simulink model "testFilter"  (R2026b)
settings: Solver=VariableStepAuto
model workspace (MAT data in the model file):
  a = 0.1
  b = 0.9
settings Model: ParameterArgumentNames=a,b  Creator=grouleau  LastModifiedBy=grouleau

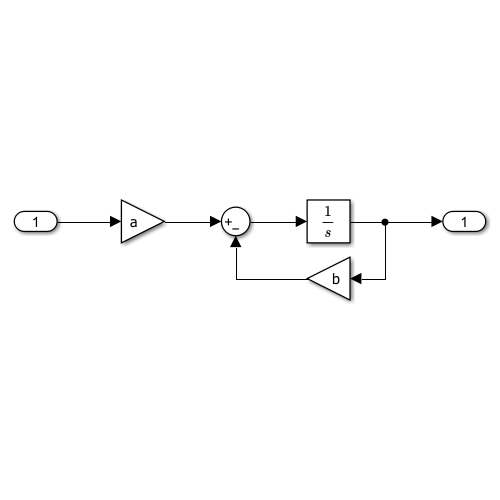
[thumbnail: Simulink's stored preview of the top-level diagram]
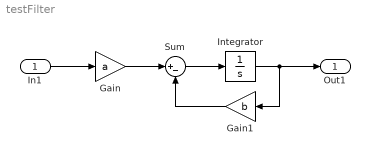
== system testFilter ==
  In1 : Inport
  Gain : Gain  Gain=a
  Gain1 : Gain  Gain=b
  Integrator : Integrator
  Sum : Sum  Inputs=|+-
  Out1 : Outport
  wires:
  In1/1 -> Gain/1
  Gain/1 -> Sum/1
  Sum/1 -> Integrator/1
  Integrator/1 -> Out1/1, Gain1/1
  Gain1/1 -> Sum/2
